simulink model "lab4_pitch"  (R2025b)
settings: Solver=FixedStepDiscrete  StartTime=0.0  StopTime=200  FixedStep=h  RelTol=1e-3
undefined symbols (not defined in the file): Ah, Aobs, Bh, Bobs, Ck, Cobs, Dobs, h, Q, R
settings Model: Creator=Nickolay  LastModifiedBy=Nickolay

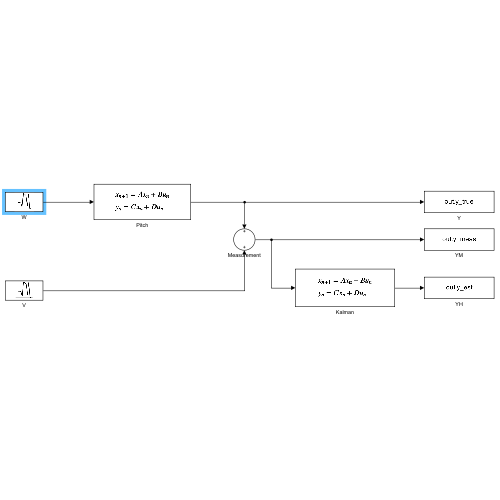
[thumbnail: Simulink's stored preview of the top-level diagram]
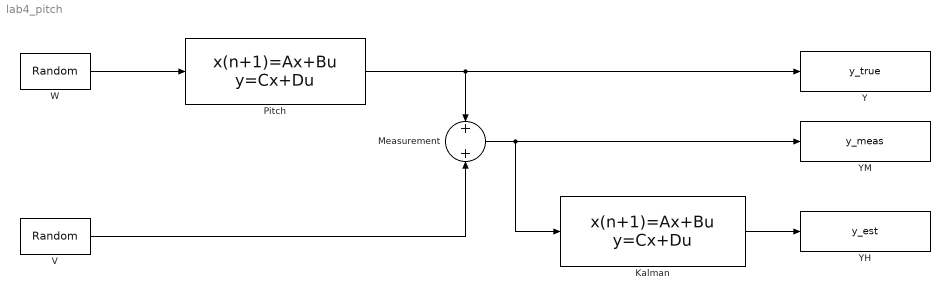
== system lab4_pitch ==
  Kalman : DiscreteStateSpace  A=Aobs  B=Bobs  C=Cobs  D=Dobs  InitialCondition=[0;0]  SampleTime=h
  Measurement : Sum
  Pitch : DiscreteStateSpace  A=Ah  B=Bh  C=Ck  D=0  InitialCondition=[0;0]  SampleTime=h
  V : RandomNumber  Variance=R  Seed=102  SampleTime=h
  W : RandomNumber  Variance=Q  Seed=101  SampleTime=h
  Y : ToWorkspace  VariableName=y_true  SaveFormat=Timeseries  SampleTime=-1
  YH : ToWorkspace  VariableName=y_est  SaveFormat=Timeseries  SampleTime=-1
  YM : ToWorkspace  VariableName=y_meas  SaveFormat=Timeseries  SampleTime=-1
  wires:
  W/1 -> Pitch/1
  Pitch/1 -> Measurement/1, Y/1
  V/1 -> Measurement/2
  Measurement/1 -> YM/1, Kalman/1
  Kalman/1 -> YH/1
